simulink model "UHG_PID_control_5"  (R2023a)
settings: Solver=VariableStepAuto  StartTime=0.0  StopTime=150  RelTol=1e-3
model workspace (MAT data in the model file):
  TimeStep = Simulink.Parameter
  TimeStep.Value = 0.01
  TimeStep.DataType = 'auto'
  TimeStep.Complexity = 'real'
  TimeStep.Dimensions = [1 1]
libraries: slctrlblks x1, slpidlib x1, simulink x1, SignalEditorBlockLib x1
settings Model: Creator=tshintai  LastModifiedBy=tshintai
settings SolverCC: AlgebraicLoopSolver=TrustRegion
settings OptimizationCC: ReuseModelBlockBuffer=off
settings DebuggingCC: UnconnectedInputMsg=warning  UnconnectedOutputMsg=warning  UnconnectedLineMsg=warning
settings ModelReferenceCC: EnableRefExpFcnMdlSchedulingChecks=on
settings RTWCC: DLArmComputeVersion=19.05

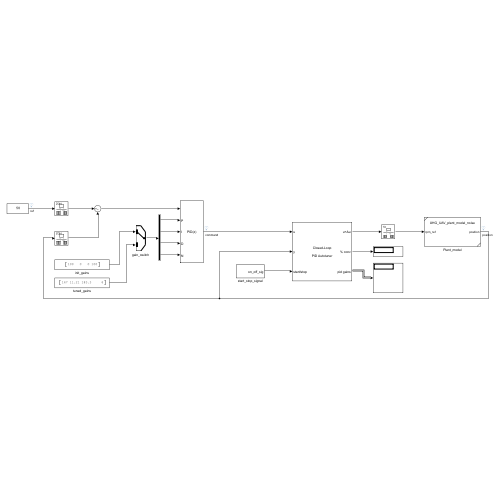
[thumbnail: Simulink's stored preview of the top-level diagram]
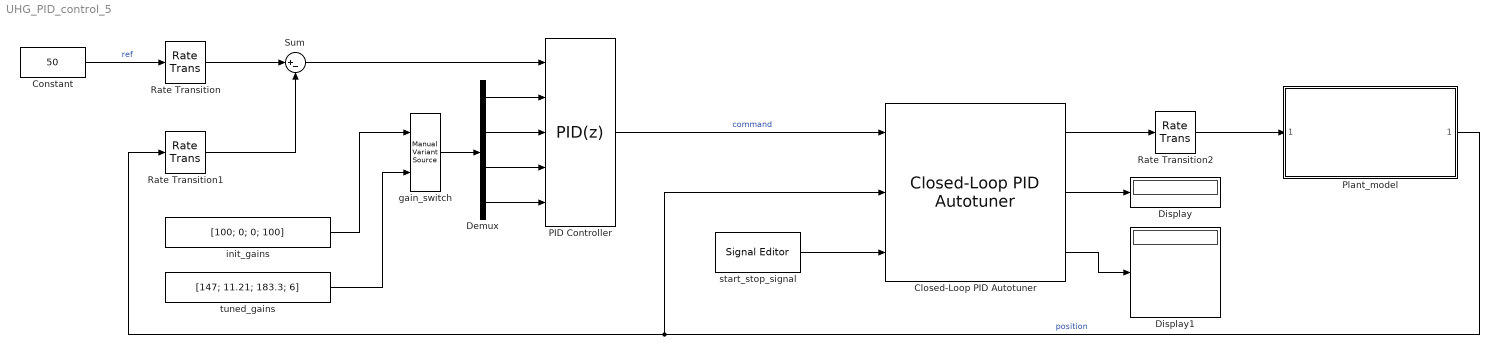
== system UHG_PID_control_5 ==
  Closed-Loop PID Autotuner : slctrlblks/Closed-Loop PID Autotuner  PIDType=PIDF  PIDForm=Parallel  TimeDomain=discrete-time  DiscreteTs=TimeStep  TuningTs=0.2  UseTuningTs=off  IntegratorFormula=Forward Euler  FilterFormula=Forward Euler  ContinuousTs=0.02  Bandwidth=2  UseExternalWC=off  TargetPM=60  UseExternalPM=off  UseExternalAchievedPM=off  ExperimentMode=Superposition  PlantType=Integrating  PlantSign=Positive  AmpSine=200  UseExternalAmpSine=off  UseExternalFRD=off  UseExternalU0=off  UseCompanion=off  NotDeployTuningModule=off  UsePLCCoder=off  OutputMode=control action + perturbation  BlockDataType=double  UseConnectedPID=on  blockpath=[]  tunedP=0  tunedI=0  tunedD=0  tunedN=100  tunedPM=0  EstimationWindowSize=3  UseExternalTuningParams=off  SingleMultiRateVariant=SingleSamplingRate  NumEstimationPeriods=4  NumSettlingPeriods=2  ExperimentModeVariant=VariantSuperimposed  OutputChoice=VariantCandD
  Constant : Constant  Value=50
  Demux : Demux
  Display : Display
  Display1 : Display
  PID Controller : slpidlib/PID Controller  Controller=PID  Form=Parallel  TimeDomain=Discrete-time  UseExternalTs=off  SampleTime=TimeStep  IntegratorMethod=Forward Euler  FilterMethod=Forward Euler  ControllerParametersSource=external  P=0  I=0  UseKiTs=off  D=0  N=3  UseFilter=on  TunerSelectOption=Transfer Function Based (PID Tuner App)  InitialConditionSource=internal  InitialConditionForIntegrator=0  InitialConditionForFilter=0  DifferentiatorICPrevScaledInput=0  ExternalReset=none  TrackingMode=off  Kt=1  LimitOutput=off  SatLimitsSource=internal  UpperSaturationLimit=inf  LowerSaturationLimit=-inf  LinearizeAsGain=on  AntiWindupMode=none  Kb=1  LimitIntegrator=off  UpperIntegratorSaturationLimit=inf  LowerIntegratorSaturationLimit=-inf  POutMin=[]  POutMax=[]  IOutMin=[]  IOutMax=[]  DOutMin=[]  DOutMax=[]  NOutMin=[]  NOutMax=[]  SumOutMin=[]  SumOutMax=[]  SaturationOutMin=[]  SaturationOutMax=[]  PParamMin=[]  PParamMax=[]  IParamMin=[]  IParamMax=[]  DParamMin=[]  DParamMax=[]  NParamMin=[]  NParamMax=[]  KbParamMin=[]  KbParamMax=[]  KtParamMin=[]  KtParamMax=[]  KbOutMin=[]  KbOutMax=[]  KtOutMin=[]  KtOutMax=[]  IntegratorOutMin=[]  IntegratorOutMax=[]  FilterOutMin=[]  FilterOutMax=[]  SumI1OutMin=[]  SumI1OutMax=[]  SumI2OutMin=[]  SumI2OutMax=[]  SumI3OutMin=[]  SumI3OutMax=[]  SumI4OutMin=[]  SumI4OutMax=[]  SumDOutMin=[]  SumDOutMax=[]  DifferentiatorOutMin=[]  DifferentiatorOutMax=[]  FilterDiffOutCoefMin=[]  FilterDiffOutCoefMax=[]  ReciprocalOutMin=[]  ReciprocalOutMax=[]  SumDenOutMin=[]  SumDenOutMax=[]  SumNumOutMin=[]  SumNumOutMax=[]  DivideOutMin=[]  DivideOutMax=[]  UdiffTsProdOutMin=[]  UdiffTsProdOutMax=[]  NTsProdOutMin=[]  NTsProdOutMax=[]  UintegralTsProdOutMin=[]  UintegralTsProdOutMax=[]  UngainTsProdOutMin=[]  UngainTsProdOutMax=[]  ClampingZeroOutDataTypeStr=Inherit: Inherit via back propagation  ClampingZeroOutMin=[]  ClampingZeroOutMax=[]  FilterDenConstantOutDataTypeStr=Inherit: Inherit via back propagation  FilterDenConstantOutMin=[]  FilterDenConstantOutMax=[]  PCopyOutDataTypeStr=Inherit: Inherit via back propagation  PCopyOutMin=[]  PCopyOutMax=[]  NCopyOutDataTypeStr=Inherit: Inherit via back propagation  NCopyOutMin=[]  NCopyOutMax=[]  IntegratorContinuousStateAttributes=''  IntegratorStateMustResolveToSignalObject=off  IntegratorRTWStateStorageClass=Auto  FilterContinuousStateAttributes=''  FilterStateMustResolveToSignalObject=off  FilterRTWStateStorageClass=Auto  ParallelPVariant=ExternalParameters  IdealPVariant=Disabled  IVariant=ExternalParameters  DVariant=ExternalParameters  IntegratorVariant=Discrete  SatVariant=Disabled  AWVariant=Passthrough  PCopyVariant=Disabled  TRVariant=Disabled  FdbkBlocksVariant=Forward  IdealPFdbkVariant=Disabled  SatFdbkVariant=Disabled  DerivativeFilterVariant=ForwardEulerFilter  NVariant=ExternalParameters  NCopyVariant=Disabled  FilterICVariant=InternalICsFilter  IntegratorICVariant=InternalICs  ExternalResetVariant=Disabled  TRSumVariant=Passthrough  SumFdbkVariant=Disabled  SumVariant=Sum_PID  TsampFilterVariant=InternalTs  TsampNgainVariant=Passthrough  TsampIntegralVariant=Disabled_SignalSpec  ExternalSaturationOutDataTypeStr=Inherit: Same as second input
  Plant_model : Subsystem  ReferencedSubsystem=UHG_UAV_plant_model_noise
  Rate Transition : RateTransition  OutPortSampleTime=TimeStep
  Rate Transition1 : RateTransition  OutPortSampleTime=TimeStep
  Rate Transition2 : RateTransition
  Sum : Sum  Inputs=|+-
  gain_switch : simulink/Signal Routing/Manual Variant Source  NumChoices=2  LabelModeActiveChoice=V_1
  init_gains : Constant  Value=[100; 0; 0; 100]
  start_stop_signal : SignalEditorBlockLib/Signal Editor  FileName=UHG_PID_control_5_signal.mat  ActiveScenario=No_op  ActiveSignal=on_off_sig  IsBus=off  OutputBusObjectStr=Bus: BusObject  SampleTime=TimeStep  Interpolate=off  ZeroCross=off  OutputAfterFinalValue=Holding final value  Unit=inherit  PreserveSignalName=on  ApplySigPropsToAllScenarios=on
  tuned_gains : Constant  Value=[147; 11.21; 183.3; 6]
  wires:
  Sum/1 -> PID Controller/1
  Constant/1 -> Rate Transition/1  "ref"
  Plant_model/1 -> Rate Transition1/1, Closed-Loop PID Autotuner/2  "position"
  PID Controller/1 -> Closed-Loop PID Autotuner/1  "command"
  Closed-Loop PID Autotuner/1 -> Rate Transition2/1
  Rate Transition/1 -> Sum/1
  Rate Transition1/1 -> Sum/2
  start_stop_signal/1 -> Closed-Loop PID Autotuner/3
  Closed-Loop PID Autotuner/2 -> Display/1
  Closed-Loop PID Autotuner/3 -> Display1/1
  Rate Transition2/1 -> Plant_model/1
  Demux/1 -> PID Controller/2
  Demux/2 -> PID Controller/3
  Demux/3 -> PID Controller/4
  Demux/4 -> PID Controller/5
  gain_switch/1 -> Demux/1
  init_gains/1 -> gain_switch/1
  tuned_gains/1 -> gain_switch/2
